simulink model "FeedbackControl_MVP_AI"  (R2026b)
settings: Solver=ode4  StopTime=90  FixedStep=0.005
settings Model: DataDictionary=QuadInterfaces_AI.sldd  Creator=JonathanTee  LastModifiedBy=JonathanTee

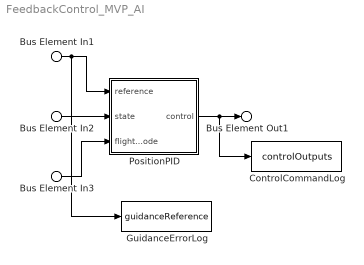
== system FeedbackControl_MVP_AI ==
  Bus Element In1 : Inport  PortName=PositionReference
  Bus Element In2 : Inport  Port=2  PortName=VehicleState
  Bus Element In3 : Inport  Port=3  PortName=FlightMode
  ControlCommandLog : ToWorkspace  VariableName=controlOutputs  SaveFormat=Timeseries  SampleTime=-1
  GuidanceErrorLog : ToWorkspace  VariableName=guidanceReference  SaveFormat=Timeseries  SampleTime=-1
  PositionPID : MATLAB Function  TreatAsAtomicUnit=on
  Bus Element Out1 : Outport  PortName=ControlOutputs
  wires:
  Bus Element In3/1 -> PositionPID/3(flightMode)
  Bus Element In2/1 -> PositionPID/2(state)
  Bus Element In1/1 -> GuidanceErrorLog/1, PositionPID/1(reference)
  PositionPID/1(control) -> ControlCommandLog/1, Bus Element Out1/1

== matlab function FeedbackControl_MVP_AI/PositionPID ==
  settings: updateMethod=DISCRETE  sampleTime=MVP.SampleTime
  data: reference input Bus: PositionReference_IF; control output Bus: ControlOutputs_IF; state input Bus: VehicleState_IF; flightMode input Bus: FlightMode_IF
function control=feedback(reference,state,flightMode)
%#codegen
control=stage02_feedback_control(reference,state,flightMode);
end
